simulink model "ECM_1RC_battery_table_based"  (R2025b)
settings: Solver=ode23t  StartTime=0.0  StopTime=4500  MaxStep=0.1  RelTol=1e-3
libraries: nesl_utility x4, fl_lib x3, batteryecm_lib x1, simulink x1
settings Model: Creator=SAT  LastModifiedBy=SAT

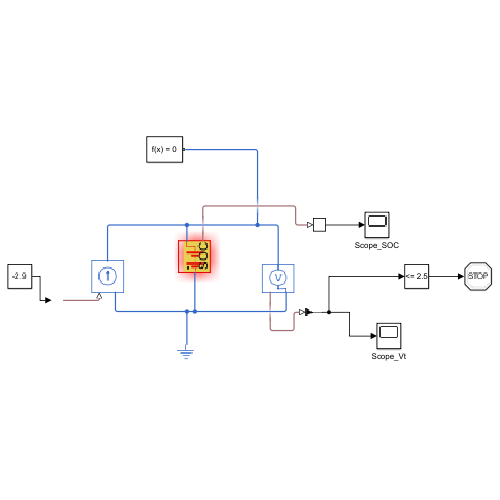
[thumbnail: Simulink's stored preview of the top-level diagram]
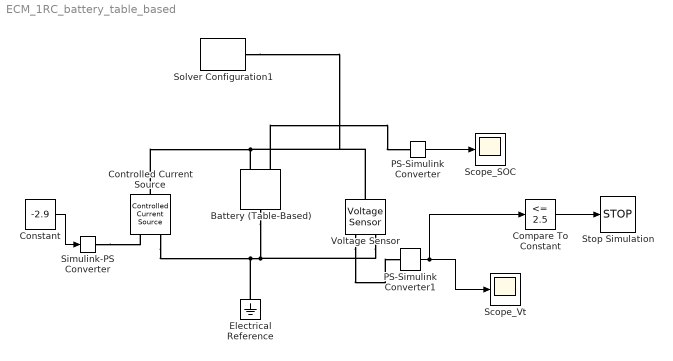
== system ECM_1RC_battery_table_based ==
  Battery (Table-Based) : batteryecm_lib/Battery (Table-Based)  SOC_vec=SOC_vec  T_dependence=simscape.enum.tablebattery.temperature_dependence.no  prm_dir=simscape.enum.tablebattery.prm_dir.noCurrentDirectionality  T_vec=[278, 293, 313] K  V0_mat=[3.49, 3.5, 3.51; 3.55, 3.57, 3.56; 3.62, 3.63, 3.64; 3.71, 3.71, 3.72; 3.91, 3.93, 3.94; 4.07, 4.08, 4.08; 4.19, 4.19, 4.19] V  V0_vec=OCV_vec V  V_range="[2.0 4.3]  V"  R0_mat=[.0117, .0085, .009; .011, .0085, .009; .0114, .0087, .0092; .0107, .0082, .0088; .0107, .0083, .0091; .0113, .0085, .0089; .0116, .0085, .0089] Ohm  R0_vec=R0_vec Ohm  R0_dis_mat=[.0117, .0085, .009; .011, .0085, .009; .0114, .0087, .0092; .0107, .0082, .0088; .0107, .0083, .0091; .0113, .0085, .0089; .0116, .0085, .0089] Ohm  R0_dis_vec=[.0085, .0085, .0087, .0082, .0083, .0085, .0085] Ohm  R0_ch_mat=[.0117, .0085, .009; .011, .0085, .009; .0114, .0087, .0092; .0107, .0082, .0088; .0107, .0083, .0091; .0113, .0085, .0089; .0116, .0085, .0089] Ohm  R0_ch_vec=[.0085, .0085, .0087, .0082, .0083, .0085, .0085] Ohm  AH=Cap_Ah A*hr  prm_leak=simscape.enum.tablebattery.prm_leak.disabled  Rleak_vec=[8000, 7000, 6000] Ohm  Rleak=7e3 Ohm  extrapolation_option=simscape.enum.extrapolation.nearest  SOC_port=simscape.enum.tablebattery.enable.yes  prm_dyn=simscape.enum.tablebattery.prm_dyn.rc1  R1_mat=[.0109, .0029, .0013; .0069, .0024, .0012; .0047, .0026, .0013; .0034, .0016, .001; .0033, .0023, .0014; .0033, .0018, .0011; .0028, .0017, .0011] Ohm  R1_vec=R1_vec Ohm  tau1_mat=[20, 36, 39; 31, 45, 39; 109, 105, 61; 36, 29, 26; 59, 77, 67; 40, 33, 29; 25, 39, 33] s  tau1_vec=tau1_vec s  R2_mat=[.0109, .0029, .0013; .0069, .0024, .0012; .0047, .0026, .0013; .0034, .0016, .001; .0033, .0023, .0014; .0033, .0018, .0011; .0028, .0017, .0011] Ohm  R2_vec=[.0029, .0024, .0026, .0016, .0023, .0018, .0017] Ohm  tau2_mat=[20, 36, 39; 31, 45, 39; 109, 105, 61; 36, 29, 26; 59, 77, 67; 40, 33, 29; 25, 39, 33] s  tau2_vec=[36, 45, 105, 29, 77, 33, 39] s  R3_mat=[.0109, .0029, .0013; .0069, .0024, .0012; .0047, .0026, .0013; .0034, .0016, .001; .0033, .0023, .0014; .0033, .0018, .0011; .0028, .0017, .0011] Ohm  R3_vec=[.0029, .0024, .0026, .0016, .0023, .0018, .0017] Ohm  tau3_mat=[20, 36, 39; 31, 45, 39; 109, 105, 61; 36, 29, 26; 59, 77, 67; 40, 33, 29; 25, 39, 33] s  tau3_vec=[36, 45, 105, 29, 77, 33, 39] s  R4_mat=[.0109, .0029, .0013; .0069, .0024, .0012; .0047, .0026, .0013; .0034, .0016, .001; .0033, .0023, .0014; .0033, .0018, .0011; .0028, .0017, .0011] Ohm  R4_vec=[.0029, .0024, .0026, .0016, .0023, .0018, .0017] Ohm  tau4_mat=[20, 36, 39; 31, 45, 39; 109, 105, 61; 36, 29, 26; 59, 77, 67; 40, 33, 29; 25, 39, 33] s  tau4_vec=[36, 45, 105, 29, 77, 33, 39] s  R5_mat=[.0109, .0029, .0013; .0069, .0024, .0012; .0047, .0026, .0013; .0034, .0016, .001; .0033, .0023, .0014; .0033, .0018, .0011; .0028, .0017, .0011] Ohm  R5_vec=[.0029, .0024, .0026, .0016, .0023, .0018, .0017] Ohm  tau5_mat=[20, 36, 39; 31, 45, 39; 109, 105, 61; 36, 29, 26; 59, 77, 67; 40, 33, 29; 25, 39, 33] s  tau5_vec=[36, 45, 105, 29, 77, 33, 39] s  prm_fade=simscape.enum.tablebattery.prm_fade.disabled  N0=100  dV0=0  dR0=0  dAH=0  dRleak=0  dR1=0  dR2=0  dR3=0  dR4=0  dR5=0  N0vec=[0, 100, 200, 300]  Tfadevec=[298.15, 323.15] K  dV0vec=[0, 0, 0, 0]  dR0vec=[0, 0, 0, 0]  dAHvec=[0, 0, 0, 0]  dRleakvec=[0, 0, 0, 0]  dR1vec=[0, 0, 0, 0]  dR2vec=[0, 0, 0, 0]  dR3vec=[0, 0, 0, 0]  dR4vec=[0, 0, 0, 0]  dR5vec=[0, 0, 0, 0]  dV0mat=[0, 0; 0, 0; 0, 0; 0, 0]  dR0mat=[0, 0; 0, 0; 0, 0; 0, 0]  dAHmat=[0, 0; 0, 0; 0, 0; 0, 0]  dRleakmat=[0, 0; 0, 0; 0, 0; 0, 0]  dR1mat=[0, 0; 0, 0; 0, 0; 0, 0]  dR2mat=[0, 0; 0, 0; 0, 0; 0, 0]  dR3mat=[0, 0; 0, 0; 0, 0; 0, 0]  dR4mat=[0, 0; 0, 0; 0, 0; 0, 0]  dR5mat=[0, 0; 0, 0; 0, 0; 0, 0]  prm_age_modeling=simscape.enum.tablebattery.prm_age_modeling.equation  storage_dt_age_vec=[0] d  storage_T_age_vec=[273] K  prm_age_OCV=simscape.enum.tablebattery.prm_age_OCV.OCV  OCV_age=0.9  SOC_age=0.6  prm_age_resistance=simscape.enum.tablebattery.prm_age.disabled  OCV_scaling_age_resistance=2.2134e6  OCV_offset_age_resistance=1.632e6  temp_exp_age_resistance=0.515833569 V  t_exp_age_resistance=0.75  T_age_vec_resistance=[273.15, 298.15, 323.15] K  dt_age_vec_resistance=[0, 90, 180, 270] d  dR0_age_vec=[0, 0, 0]  t_meas_dR0_age=100 d  dR0_age_mat=[0, 0, 0; 0, 0, 0; 0, 0, 0; 0, 0, 0]  prm_age_capacity=simscape.enum.tablebattery.prm_age.disabled  OCV_scaling_age_capacity=1.5097e07  OCV_offset_age_capacity=8.3625e06  temp_exp_age_capacity=0.6011 V  t_exp_age_capacity=0.75  T_age_vec_capacity=[273.15, 298.15, 323.15] K  dt_age_vec_capacity=[0, 90, 180, 270] d  dAH_age_vec=[0, 0, 0]  t_meas_dAH_age=100 d  dAH_age_mat=[0, 0, 0; 0, 0, 0; 0, 0, 0; 0, 0, 0]  thermal_port=simscape.enum.thermaleffects.omit  temperature=298.15 K  thermal_mass=100 J/K  i_specify=off  i_priority=None  i=0 A  i_nominal_specify=off  i_nominal_value=1  i_nominal_unit=A  v_specify=off  v_priority=None  v=0 V  v_nominal_specify=off  v_nominal_value=1  v_nominal_unit=V  stateOfCharge_specify=on  stateOfCharge_priority=High  stateOfCharge=1  stateOfCharge_nominal_specify=off  stateOfCharge_nominal_value=1  stateOfCharge_nominal_unit=1  num_cycles_specify=off  num_cycles_priority=High  num_cycles=0  num_cycles_nominal_specify=off  num_cycles_nominal_value=1  num_cycles_nominal_unit=1  cell_temperature_specify=off  cell_temperature_priority=High  cell_temperature=298.15 K  cell_temperature_nominal_specify=off  cell_temperature_nominal_value=1  cell_temperature_nominal_unit=K
      settings: InternalSimscapePortConfiguration="{\"Bottom\":[],\"Left\":[{\"id\":\"p\",\"label\":\"+\",\"type\":\"foundation.electrical.electrical\"},{\"id\":\"soc\",\"label\":\"SOC\",\"type\":\"output\"}],\"Right\":[{\"id\":\"n\",\"label\":\"-\",\"type\":\"foundation.electrical.electrical\"}],\"Top\":[]}"
      settings: LibrarySourceBlock=|
      | batt_lib/Cells/Battery
      | (Table-Based)
  Compare To Constant : simulink/Logic and Bit Operations/Compare To Constant  relop=<=  const=2.5  OutDataTypeStr=boolean
  Constant : Constant  Value=-2.9
  Controlled Current Source : fl_lib/Electrical/Electrical Sources/Controlled Current Source
  Electrical Reference : fl_lib/Electrical/Electrical Elements/Electrical Reference
  PS-Simulink Converter : nesl_utility/PS-Simulink Converter  PhysicalDomain=network_engine_domain  SubClassName=ps_output  LeftPortType=input  RightPortType=output  PseudoPeriodic=off  Frequencies=[]  VectorFormat=inherit  Unit=inherit  AffineConversion=off
  PS-Simulink Converter1 : nesl_utility/PS-Simulink Converter  PhysicalDomain=network_engine_domain  SubClassName=ps_output  LeftPortType=input  RightPortType=output  PseudoPeriodic=off  Frequencies=[]  VectorFormat=inherit  Unit=inherit  AffineConversion=off
  Scope_SOC : Scope
      settings: ActiveDisplayYMinimum=-0.12500000000004333  ActiveDisplayYMaximum=1.1250000000000049
  Scope_Vt : Scope
      settings: ActiveDisplayYMinimum=2.4047818650536081  ActiveDisplayYMaximum=4.3382590552670521
  Simulink-PS Converter : nesl_utility/Simulink-PS Converter  PhysicalDomain=network_engine_domain  SubClassName=ps_input  LeftPortType=input  RightPortType=output  PseudoPeriodic=off  Frequencies=[]  NoiseDistribution=none  NoiseParameters=[]  Unit=1  AffineConversion=off  FilteringAndDerivatives=provide  SimscapeFilterOrder=1  InputFilterTimeConstant=0.001  UdotUserProvided=0
  Solver Configuration1 : nesl_utility/Solver Configuration  PhysicalDomain=network_engine_domain  SubClassName=solver  LeftPortType=input  RightPortType=generic  Tones=[]  Harmonics=[]  SimulateNoise=off  Profile=off  UseLocalSampling=off  EnableSwitchedLinearOptims=on  FrequencyDomain=off  UseCCode=off  RelTol=0.001  AbsTol=0.001  MinStep=1e-09  ToWorkspace=off  RevertToSquareIcSolve=off  NumHomotopyIterations=100  PhasorMode=off  PhasorModeNumHarmonics=1  ConsistencySolver=NEWTON_XTOL_AFTER_FTOL  IndexReductionMethod=DerivativeReplacement  DoDC=off  ResidualTolerance=1e-09  ConsistencyTolSource=GLOBAL  ConsistencyAbsTol=0.001  ConsistencyRelTol=0.001  ConsistencyTolFactor=0.001  UseLocalSolver=on  LocalSolverChoice=NE_BACKWARD_EULER_ADVANCER  ResolveIndetEquations=on  FunctionEvalNumThread=1  LocalSolverSampleTime=0.5  DoFixedCost=off  MaxNonlinIter=3  MaxModeIter=2  ComputeImpulses=off  ImpulseIterations=2  LinearAlgebra=auto  LinearAlgebraNumThread=0  EquationFormulation=NE_TIME_EF  DelaysMemoryBudget=1024  AutomaticFiltering=on  FilteringTimeConstant=0.001  PartitionStorageMethod=AS_NEEDED  PartitionMemoryBudget=1024  PartitionMethod=ROBUST  MultibodyUseLocalSolver=off  MultibodyLocalSolverChoice=ODE1  MultibodyLocalSolverSampleTime=0.001
  Stop Simulation : Stop
  Voltage Sensor : fl_lib/Electrical/Electrical Sensors/Voltage Sensor
  wires:
  Constant/1 -> Simulink-PS Converter/1
  PS-Simulink Converter/1 -> Scope_SOC/1
  PS-Simulink Converter1/1 -> Compare To Constant/1, Scope_Vt/1
  Compare To Constant/1 -> Stop Simulation/1
  connections:
  Controlled Current Source/LConn1 -- Solver Configuration1/RConn1 -- Voltage Sensor/LConn1 -- Battery (Table-Based)/LConn1
  Controlled Current Source/RConn2 -- Electrical Reference/LConn1 -- Battery (Table-Based)/RConn1 -- Voltage Sensor/RConn2
  Simulink-PS Converter/RConn1 -- Controlled Current Source/RConn1
  Voltage Sensor/RConn1 -- PS-Simulink Converter1/LConn1
  Battery (Table-Based)/LConn2 -- PS-Simulink Converter/LConn1
